simulink model "bms_estimator_ref"  (R2024b)
settings: Solver=FixedStepDiscrete  StartTime=0.0  StopTime=10.0  FixedStep=1  RelTol=1e-3
settings Model: DataDictionary=bms_data.sldd  Creator=sande  LastModifiedBy=sande
settings DebuggingCC: SignalInfNanChecking=error  AlgebraicLoopMsg=error  ArtificialAlgebraicLoopMsg=error  UnconnectedInputMsg=error  UnconnectedOutputMsg=error  UnconnectedLineMsg=error  BusObjectLabelMismatch=error  StrictBusMsg=ErrorOnBusTreatedAsVector

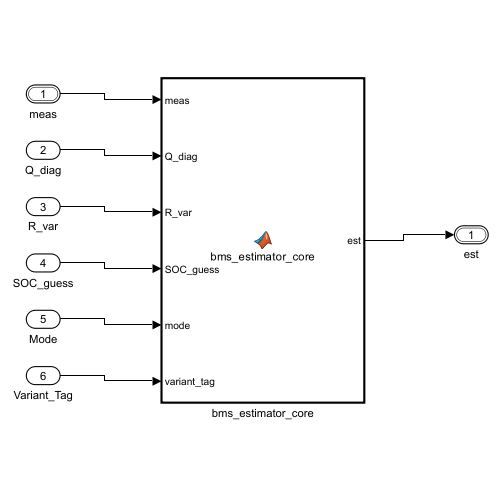
[thumbnail: Simulink's stored preview of the top-level diagram]
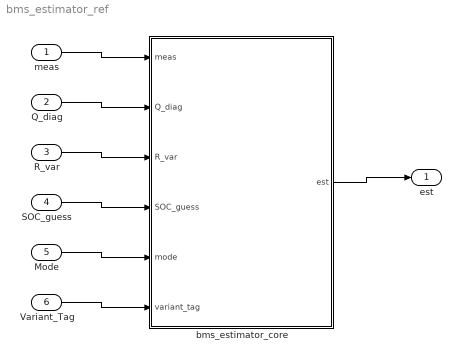
== system bms_estimator_ref ==
  meas : Inport  OutDataTypeStr=Bus: BMS_Measurement  PortDimensions=1
  Q_diag : Inport  Port=2  OutDataTypeStr=double  PortDimensions=3
  R_var : Inport  Port=3  OutDataTypeStr=double  PortDimensions=1
  SOC_guess : Inport  Port=4  OutDataTypeStr=double  PortDimensions=1
  Mode : Inport  Port=5  OutDataTypeStr=double  PortDimensions=1
  Variant_Tag : Inport  Port=6  OutDataTypeStr=double  PortDimensions=1
  bms_estimator_core : MATLAB Function  TreatAsAtomicUnit=on
  est : Outport  OutDataTypeStr=Bus: BMS_Estimate
  wires:
  meas/1 -> bms_estimator_core/1(meas)
  Q_diag/1 -> bms_estimator_core/2(Q_diag)
  R_var/1 -> bms_estimator_core/3(R_var)
  SOC_guess/1 -> bms_estimator_core/4(SOC_guess)
  Mode/1 -> bms_estimator_core/5(mode)
  Variant_Tag/1 -> bms_estimator_core/6(variant_tag)
  bms_estimator_core/1(est) -> est/1

== matlab function bms_estimator_ref/bms_estimator_core ==
  data: meas input Bus: BMS_Measurement; est output Bus: BMS_Estimate; Q_diag input; R_var input; SOC_guess input; mode input; variant_tag input
function est = bms_estimator_core(meas, Q_diag, R_var, SOC_guess, mode, variant_tag)
%#codegen
% Multi-mode 4-state Joseph-form EKF core wrapped for Model Reference.
P_syn  = coder.const(bms_params('synthetic'));
P_nasa = coder.const(bms_params('nasa'));
if variant_tag > 0.5
    P = P_nasa;
else
    P = P_syn;
end
persistent st;
if isempty(st)
    st = bms_est_init(P, SOC_guess, Q_diag, R_var, mode);
end
[st, o] = bms_est_step(st, meas.Current_A, meas.Voltage_V, meas.Temperature_K, P, mode);
est.SOC_pct = o.soc;
est.Voltage_V = o.vest;
est.Innovation_V = o.innov;
est.PTrace = o.ptrace;
est.NIS = o.nis;
est.FaultCode = o.fault;
est.R0_Ohm = o.r0;
est.SOC_Coulomb_pct = o.soc_cc;
est.R_cov_V2 = o.rcov;
est.CapacityRatio = o.cap;
